simulink model "Simscape_model_Energy"  (R2026a)
settings: Solver=FixedStepAuto  StopTime=8  FixedStep=0.0001
model workspace (MATLAB code in the model file):
  | clear; clc; close all;
values from neighbouring files (symbols this model uses):
  black = partTemplate    [Parameters.m]    (also in Parameters_optimization.m = struct)
  blueBlock = partTemplate    [Parameters.m]    (also in Parameters_optimization.m = struct)
  cyan = partTemplate    [Parameters.m]    (also in Parameters_optimization.m = struct)
  g = 9.81    [Parameters.m]    (also in Parameters_optimization.m)
  greenBeam = partTemplate    [Parameters.m]    (also in Parameters_optimization.m = struct)
  greenBlock = partTemplate    [Parameters.m]    (also in Parameters_optimization.m = struct)
  grey = partTemplate    [Parameters.m]    (also in Parameters_optimization.m = struct)
  IMax = 16    [Parameters.m]    (also in Parameters_optimization.m)
  IMin = -16    [Parameters.m]    (also in Parameters_optimization.m)
  JM = 0.002    [Parameters.m]    (also in Parameters_optimization.m)
  KdA_pos = 1    [Parameters.m]    (also in Parameters_optimization.m = 5066.74)
  KdA_vel = 0    [Parameters.m]    (also in Parameters_optimization.m)
  KdB1_pos = 1    [Parameters.m]    (also in Parameters_optimization.m = 4.04669)
  KdB1_vel = 0    [Parameters.m]    (also in Parameters_optimization.m)
  KdB2_pos = 1    [Parameters.m]    (also in Parameters_optimization.m = 1.06194)
  KdB2_vel = 0    [Parameters.m]    (also in Parameters_optimization.m)
  KdG_pos = 1    [Parameters.m]    (also in Parameters_optimization.m = 1.01282)
  KdG_vel = 0    [Parameters.m]    (also in Parameters_optimization.m)
  KdH_pos = 1    [Parameters.m]    (also in Parameters_optimization.m = 16.6487)
  KdH_vel = 0    [Parameters.m]    (also in Parameters_optimization.m)
  KdI_pos = 1    [Parameters.m]    (also in Parameters_optimization.m = 2.31436)
  KdI_vel = 0    [Parameters.m]    (also in Parameters_optimization.m)
  KiA_pos = 2    [Parameters.m]    (also in Parameters_optimization.m = 1.00755)
  KiA_vel = 5    [Parameters.m]    (also in Parameters_optimization.m)
  KiB1_pos = 30    [Parameters.m]    (also in Parameters_optimization.m = 45.4381)
  KiB1_vel = 10    [Parameters.m]    (also in Parameters_optimization.m)
  KiB2_pos = 20    [Parameters.m]    (also in Parameters_optimization.m = 84.4311)
  KiB2_vel = 5    [Parameters.m]    (also in Parameters_optimization.m)
  KiG_pos = 30    [Parameters.m]    (also in Parameters_optimization.m = 81.5274)
  KiG_vel = 5    [Parameters.m]    (also in Parameters_optimization.m)
  KiH_pos = 10    [Parameters.m]    (also in Parameters_optimization.m = 20739.8)
  KiH_vel = 0    [Parameters.m]    (also in Parameters_optimization.m)
  KiI_pos = 0    [Parameters.m]    (also in Parameters_optimization.m = 1)
  KiI_vel = 0    [Parameters.m]    (also in Parameters_optimization.m)
  KmA = 1.5    [Parameters.m]    (also in Parameters_optimization.m = 1)
  KmB1 = 1.5    [Parameters.m]    (also in Parameters_optimization.m)
  KmB2 = 1.5    [Parameters.m]    (also in Parameters_optimization.m = 1)
  KmG = 0.5    [Parameters.m]    (also in Parameters_optimization.m)
  KmH = 1    [Parameters.m]    (also in Parameters_optimization.m = 0.5)
  KmI = 0.5    [Parameters.m]    (also in Parameters_optimization.m)
  KpA_pos = 150    [Parameters.m]    (also in Parameters_optimization.m = 1588.6)
  KpA_vel = 30    [Parameters.m]    (also in Parameters_optimization.m)
  KpB1_pos = 200    [Parameters.m]    (also in Parameters_optimization.m = 698393)
  KpB1_vel = 30    [Parameters.m]    (also in Parameters_optimization.m)
  KpB2_pos = 150    [Parameters.m]    (also in Parameters_optimization.m = 504375)
  KpB2_vel = 30    [Parameters.m]    (also in Parameters_optimization.m)
  KpG_pos = 100    [Parameters.m]    (also in Parameters_optimization.m = 2817.67)
  KpG_vel = 50    [Parameters.m]    (also in Parameters_optimization.m)
  KpH_pos = 100    [Parameters.m]    (also in Parameters_optimization.m = 12634.3)
  KpH_vel = 20    [Parameters.m]    (also in Parameters_optimization.m)
  KpI_pos = 50    [Parameters.m]    (also in Parameters_optimization.m = 2283.96)
  KpI_vel = 20    [Parameters.m]    (also in Parameters_optimization.m)
  LB1 = 0.8    [Parameters.m]    (also in Parameters_optimization.m)
  LB2 = 0.3    [Parameters.m]    (also in Parameters_optimization.m)
  LB3 = 0.24    [Parameters.m]    (also in Parameters_optimization.m)
  Lblack1 = 0.2    [Parameters.m]    (also in Parameters_optimization.m)
  LC1 = 0.4    [Parameters.m]    (also in Parameters_optimization.m)
  LC2 = 0.225    [Parameters.m]    (also in Parameters_optimization.m)
  LG1 = 0.3    [Parameters.m]    (also in Parameters_optimization.m)
  LG2 = 0.8    [Parameters.m]    (also in Parameters_optimization.m)
  Lgrey1 = 1.175    [Parameters.m]    (also in Parameters_optimization.m)
  lightBlue = partTemplate    [Parameters.m]    (also in Parameters_optimization.m = struct)
  LLB1 = 0.248    [Parameters.m]    (also in Parameters_optimization.m)
  LLB2 = 0.235    [Parameters.m]    (also in Parameters_optimization.m)
  LR1 = 1.05    [Parameters.m]    (also in Parameters_optimization.m)
  LW1 = 1.05    [Parameters.m]    (also in Parameters_optimization.m)
  nA = 200    [Parameters.m]    (also in Parameters_optimization.m = 100)
  nB1 = 200    [Parameters.m]    (also in Parameters_optimization.m = 100)
  nB2 = 200    [Parameters.m]    (also in Parameters_optimization.m)
  nG = 20    [Parameters.m]    (also in Parameters_optimization.m)
  nH = 100    [Parameters.m]    (also in Parameters_optimization.m = 50)
  nI = 20    [Parameters.m]    (also in Parameters_optimization.m)
  omegaFilterA_pos = 60    [Parameters.m]    (also in Parameters_optimization.m)
  omegaFilterA_vel = 60    [Parameters.m]    (also in Parameters_optimization.m)
  omegaFilterB1_pos = 60    [Parameters.m]    (also in Parameters_optimization.m)
  omegaFilterB1_vel = 60    [Parameters.m]    (also in Parameters_optimization.m)
  omegaFilterB2_pos = 60    [Parameters.m]    (also in Parameters_optimization.m)
  omegaFilterB2_vel = 60    [Parameters.m]    (also in Parameters_optimization.m)
  omegaFilterG_pos = 60    [Parameters.m]    (also in Parameters_optimization.m)
  omegaFilterG_vel = 60    [Parameters.m]    (also in Parameters_optimization.m)
  omegaFilterH_pos = 60    [Parameters.m]    (also in Parameters_optimization.m)
  omegaFilterH_vel = 60    [Parameters.m]    (also in Parameters_optimization.m)
  omegaFilterI_pos = 60    [Parameters.m]    (also in Parameters_optimization.m)
  omegaFilterI_vel = 60    [Parameters.m]    (also in Parameters_optimization.m)
  red = partTemplate    [Parameters.m]    (also in Parameters_optimization.m = struct)
  trajCoeff = coeff    [Parameters.m]    (also in Parameters_optimization.m = [2000 500 1600; Path_Planning_Robot.m)
  trajTime = t    [Parameters.m]    (also in Parameters_optimization.m = [0 2 4 6 8]; Path_Planning_Robot.m)
  w = 0.1    [Parameters.m]    (also in Parameters_optimization.m)
  white = partTemplate    [Parameters.m]    (also in Parameters_optimization.m = struct)
undefined symbols (not defined in the file or in its folder): X, Y, Z
libraries: sm_lib x102, nesl_utility x58, simulink x1
(part 4 of 4)

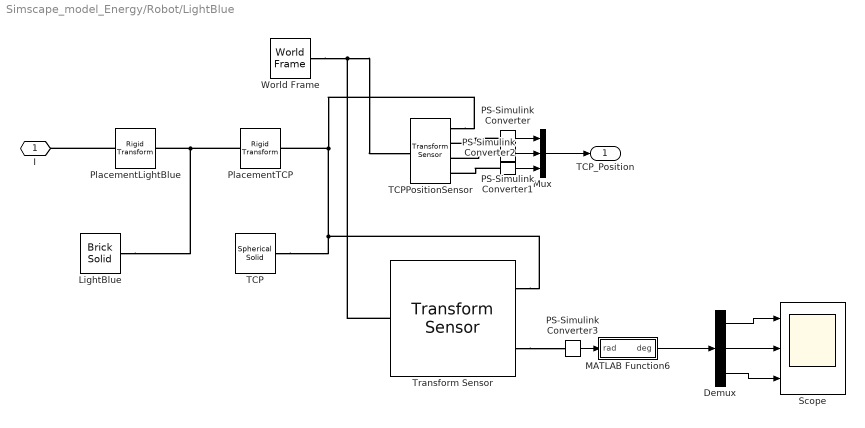
== system Simscape_model_Energy/Robot/LightBlue ==
  Demux : Demux  Outputs=3
  LightBlue : sm_lib/Body Elements/Brick Solid  BrickDimensions=[LLB2 LLB1 LLB1]  BrickDimensionsUnits=m  ExportEntireGeometry=off  InertiaType=Custom  BasedOnType=Density  Density=1000  DensityUnits=kg/m^3  Mass=lightBlue.m  MassUnits=kg  CenterOfMass=[0 0 0]  CenterOfMassUnits=m  MomentsOfInertia=[lightBlue.Ix lightBlue.Iy lightBlue.Iz]  MomentsOfInertiaUnits=kg*m^2  ProductsOfInertia=[0 0 0]  ProductsOfInertiaUnits=kg*m^2  GraphicType=FromGeometry  MarkerShape=Sphere  MarkerSize=10  GraphicVisPropType=SimpleVisualProperties  GraphicDiffuseColor=[0.6667 1 1]  GraphicOpacity=1  GraphicSpecularColor=[0.5 0.5 0.5 1.0]  GraphicAmbientColor=[0.15 0.15 0.15 1.0]  GraphicEmissiveColor=[0.0 0.0 0.0 1.0]  GraphicShininess=75  DoExposeReferenceFrame=on  SerializedFrames=<Frames/>
  MATLAB Function6 : MATLAB Function  TreatAsAtomicUnit=on
  Mux : Mux  Inputs=3
  PS-Simulink Converter{,1..3} (4 alike) : nesl_utility/PS-Simulink Converter  PhysicalDomain=network_engine_domain  SubClassName=ps_output  LeftPortType=input  RightPortType=output  PseudoPeriodic=off  Frequencies=[]  VectorFormat=inherit  Unit=inherit  AffineConversion=off
  PlacementLightBlue : sm_lib/Frames and Transforms/Rigid Transform  RotationMethod=RotationSequence  FollAlignAxisA=+X  BaseAlignAxisA=+Y  FollAlignAxisB=+Y  BaseAlignAxisB=+Z  RotationStandardAxis=+Z  RotationAngle=0  RotationAngleUnits=deg  RotationArbitraryAxis=[0 0 1]  RotationSequenceAxes=FollowerAxes  RotationSequence=XYZ  RotationSequenceAngles=[90 0 90]  RotationSequenceAnglesUnits=deg  RotationMatrix=[1 0 0;0 1 0;0 0 1]  Quaternion=[1 0 0 0]  TranslationMethod=Cartesian  TranslationCartesianOffset=[0 LLB1/2 LLB2/2]  TranslationCartesianOffsetUnits=m  TranslationStandardAxis=+Z  TranslationStandardOffset=0  TranslationStandardOffsetUnits=m  TranslationROffset=0  TranslationROffsetUnits=m  TranslationThetaOffset=0  TranslationThetaOffsetUnits=deg  TranslationZOffset=0  TranslationZOffsetUnits=m
  PlacementTCP : sm_lib/Frames and Transforms/Rigid Transform  RotationMethod=None  FollAlignAxisA=+X  BaseAlignAxisA=+Y  FollAlignAxisB=+Y  BaseAlignAxisB=+Z  RotationStandardAxis=+Z  RotationAngle=0  RotationAngleUnits=deg  RotationArbitraryAxis=[0 0 1]  RotationSequenceAxes=FollowerAxes  RotationSequence=XYZ  RotationSequenceAngles=[0 0 0]  RotationSequenceAnglesUnits=deg  RotationMatrix=[1 0 0;0 1 0;0 0 1]  Quaternion=[1 0 0 0]  TranslationMethod=Cartesian  TranslationCartesianOffset=[LLB1/2 0 -LLB2/2]  TranslationCartesianOffsetUnits=m  TranslationStandardAxis=+Z  TranslationStandardOffset=0  TranslationStandardOffsetUnits=m  TranslationROffset=0  TranslationROffsetUnits=m  TranslationThetaOffset=0  TranslationThetaOffsetUnits=deg  TranslationZOffset=0  TranslationZOffsetUnits=m
  Scope : Scope  NumInputPorts=3
      settings: ActiveDisplayYMinimum=-0.24123535125414011  ActiveDisplayYMaximum=0.21681941956598327  DataLoggingVariableName=ScopeData9
  TCP : sm_lib/Body Elements/Spherical Solid  SphereRadius=w  SphereRadiusUnits=m  ExportEntireGeometry=off  InertiaType=CalculateFromGeometry  BasedOnType=Mass  Density=0  DensityUnits=kg/m^3  Mass=0  MassUnits=kg  CenterOfMass=[0 0 0]  CenterOfMassUnits=m  MomentsOfInertia=[1 1 1]  MomentsOfInertiaUnits=kg*m^2  ProductsOfInertia=[0 0 0]  ProductsOfInertiaUnits=kg*m^2  GraphicType=FromGeometry  MarkerShape=Sphere  MarkerSize=10  GraphicVisPropType=SimpleVisualProperties  GraphicDiffuseColor=[1 0 1]  GraphicOpacity=1  GraphicSpecularColor=[0.5 0.5 0.5 1.0]  GraphicAmbientColor=[0.15 0.15 0.15 1.0]  GraphicEmissiveColor=[0.0 0.0 0.0 1.0]  GraphicShininess=75  DoExposeReferenceFrame=on  SerializedFrames=<Frames/>
  TCPPositionSensor : sm_lib/Frames and Transforms/Transform Sensor  MeasurementFrame=World  RotationSequence=XYX  SenseAngle=off  SenseAxis=off  SenseQ=off  SenseR=off  SenseRotationSequence=off  SenseOmegaX=off  SenseOmegaY=off  SenseOmegaZ=off  SenseOmega=off  SenseQDot=off  SenseRDot=off  SenseRotationSequenceDot=off  SenseAlphaX=off  SenseAlphaY=off  SenseAlphaZ=off  SenseAlpha=off  SenseQDDot=off  SenseRDDot=off  SenseX=on  SenseY=on  SenseZ=on  SenseXYZ=off  SenseRad=off  SenseAzim=off  SenseDist=off  SenseInc=off  SenseXDot=off  SenseYDot=off  SenseZDot=off  SenseXYZDot=off  SenseRadDot=off  SenseAzimDot=off  SenseDistDot=off  SenseIncDot=off  SenseXDDot=off  SenseYDDot=off  SenseZDDot=off  SenseXYZDDot=off  SenseRadDDot=off  SenseAzimDDot=off  SenseDistDDot=off  SenseIncDDot=off
  Transform Sensor : sm_lib/Frames and Transforms/Transform Sensor  MeasurementFrame=World  RotationSequence=XYZ  SenseAngle=off  SenseAxis=off  SenseQ=off  SenseR=off  SenseRotationSequence=on  SenseOmegaX=off  SenseOmegaY=off  SenseOmegaZ=off  SenseOmega=off  SenseQDot=off  SenseRDot=off  SenseRotationSequenceDot=off  SenseAlphaX=off  SenseAlphaY=off  SenseAlphaZ=off  SenseAlpha=off  SenseQDDot=off  SenseRDDot=off  SenseX=off  SenseY=off  SenseZ=off  SenseXYZ=off  SenseRad=off  SenseAzim=off  SenseDist=off  SenseInc=off  SenseXDot=off  SenseYDot=off  SenseZDot=off  SenseXYZDot=off  SenseRadDot=off  SenseAzimDot=off  SenseDistDot=off  SenseIncDot=off  SenseXDDot=off  SenseYDDot=off  SenseZDDot=off  SenseXYZDDot=off  SenseRadDDot=off  SenseAzimDDot=off  SenseDistDDot=off  SenseIncDDot=off
  World Frame : sm_lib/Frames and Transforms/World Frame
  I : PMIOPort  Side=Left
  TCP_Position : Outport
  wires:
  PS-Simulink Converter2/1 -> Mux/3
  PS-Simulink Converter1/1 -> Mux/2
  PS-Simulink Converter/1 -> Mux/1
  Mux/1 -> TCP_Position/1
  PS-Simulink Converter3/1 -> MATLAB Function6/1(rad)
  Demux/1 -> Scope/1
  Demux/2 -> Scope/2
  Demux/3 -> Scope/3
  MATLAB Function6/1(deg) -> Demux/1
  connections:
  TCP/RConn1 -- TCPPositionSensor/RConn1 -- PlacementTCP/RConn1 -- Transform Sensor/RConn1
  LightBlue/RConn1 -- PlacementTCP/LConn1 -- PlacementLightBlue/RConn1
  PlacementLightBlue/LConn1 -- I/RConn1
  PS-Simulink Converter/LConn1 -- TCPPositionSensor/RConn2
  PS-Simulink Converter1/LConn1 -- TCPPositionSensor/RConn3
  PS-Simulink Converter2/LConn1 -- TCPPositionSensor/RConn4
  World Frame/RConn1 -- Transform Sensor/LConn1 -- TCPPositionSensor/LConn1
  Transform Sensor/RConn2 -- PS-Simulink Converter3/LConn1

== system Simscape_model_Energy/Robot/Red ==
  PlacementJ3 : sm_lib/Frames and Transforms/Rigid Transform  RotationMethod=None  FollAlignAxisA=+X  BaseAlignAxisA=+Y  FollAlignAxisB=+Y  BaseAlignAxisB=+Z  RotationStandardAxis=+Z  RotationAngle=0  RotationAngleUnits=deg  RotationArbitraryAxis=[0 0 1]  RotationSequenceAxes=FollowerAxes  RotationSequence=XYX  RotationSequenceAngles=[0 0 0]  RotationSequenceAnglesUnits=deg  RotationMatrix=[1 0 0;0 1 0;0 0 1]  Quaternion=[1 0 0 0]  TranslationMethod=Cartesian  TranslationCartesianOffset=[-LR1/2 0 0]  TranslationCartesianOffsetUnits=m  TranslationStandardAxis=+Z  TranslationStandardOffset=0  TranslationStandardOffsetUnits=m  TranslationROffset=0  TranslationROffsetUnits=m  TranslationThetaOffset=0  TranslationThetaOffsetUnits=deg  TranslationZOffset=0  TranslationZOffsetUnits=m
  PlacementRed : sm_lib/Frames and Transforms/Rigid Transform  RotationMethod=RotationSequence  FollAlignAxisA=+X  BaseAlignAxisA=+Y  FollAlignAxisB=+Y  BaseAlignAxisB=+Z  RotationStandardAxis=+Z  RotationAngle=0  RotationAngleUnits=deg  RotationArbitraryAxis=[0 0 1]  RotationSequenceAxes=FollowerAxes  RotationSequence=XYZ  RotationSequenceAngles=[0 0 -90]  RotationSequenceAnglesUnits=deg  RotationMatrix=[1 0 0;0 1 0;0 0 1]  Quaternion=[1 0 0 0]  TranslationMethod=Cartesian  TranslationCartesianOffset=[-LR1/2 0 0]  TranslationCartesianOffsetUnits=m  TranslationStandardAxis=+Z  TranslationStandardOffset=0  TranslationStandardOffsetUnits=m  TranslationROffset=0  TranslationROffsetUnits=m  TranslationThetaOffset=0  TranslationThetaOffsetUnits=deg  TranslationZOffset=0  TranslationZOffsetUnits=m
  Red : sm_lib/Body Elements/Brick Solid  BrickDimensions=[LR1 w w]  BrickDimensionsUnits=m  ExportEntireGeometry=off  InertiaType=Custom  BasedOnType=Density  Density=1000  DensityUnits=kg/m^3  Mass=red.m  MassUnits=kg  CenterOfMass=[0 0 0]  CenterOfMassUnits=m  MomentsOfInertia=[red.Ix red.Iy red.Iz]  MomentsOfInertiaUnits=kg*m^2  ProductsOfInertia=[0 0 0]  ProductsOfInertiaUnits=kg*m^2  GraphicType=FromGeometry  MarkerShape=Sphere  MarkerSize=10  GraphicVisPropType=SimpleVisualProperties  GraphicDiffuseColor=[1 0 0]  GraphicOpacity=1  GraphicSpecularColor=[0.5 0.5 0.5 1.0]  GraphicAmbientColor=[0.15 0.15 0.15 1.0]  GraphicEmissiveColor=[0.0 0.0 0.0 1.0]  GraphicShininess=75  DoExposeReferenceFrame=on  SerializedFrames=<Frames/>
  E : PMIOPort  Side=Left
  B : PMIOPort  Port=2  Side=Right
  connections:
  B/RConn1 -- PlacementRed/RConn1
  PlacementRed/LConn1 -- PlacementJ3/RConn1 -- Red/RConn1
  E/RConn1 -- PlacementJ3/LConn1

== system Simscape_model_Energy/Robot/Subsystem ==
  PlacementF : sm_lib/Frames and Transforms/Rigid Transform  RotationMethod=None  FollAlignAxisA=+X  BaseAlignAxisA=+Y  FollAlignAxisB=+Y  BaseAlignAxisB=+Z  RotationStandardAxis=+Z  RotationAngle=0  RotationAngleUnits=deg  RotationArbitraryAxis=[0 0 1]  RotationSequenceAxes=FollowerAxes  RotationSequence=XYX  RotationSequenceAngles=[0 0 0]  RotationSequenceAnglesUnits=deg  RotationMatrix=[1 0 0;0 1 0;0 0 1]  Quaternion=[1 0 0 0]  TranslationMethod=Cartesian  TranslationCartesianOffset=[LW1/2 0 0]  TranslationCartesianOffsetUnits=m  TranslationStandardAxis=+Z  TranslationStandardOffset=0  TranslationStandardOffsetUnits=m  TranslationROffset=0  TranslationROffsetUnits=m  TranslationThetaOffset=0  TranslationThetaOffsetUnits=deg  TranslationZOffset=0  TranslationZOffsetUnits=m
  PlacementWhite : sm_lib/Frames and Transforms/Rigid Transform  RotationMethod=RotationSequence  FollAlignAxisA=+X  BaseAlignAxisA=+Y  FollAlignAxisB=+Y  BaseAlignAxisB=+Z  RotationStandardAxis=+Z  RotationAngle=0  RotationAngleUnits=deg  RotationArbitraryAxis=[0 0 1]  RotationSequenceAxes=FollowerAxes  RotationSequence=XYZ  RotationSequenceAngles=[0 0 90]  RotationSequenceAnglesUnits=deg  RotationMatrix=[1 0 0;0 1 0;0 0 1]  Quaternion=[1 0 0 0]  TranslationMethod=Cartesian  TranslationCartesianOffset=[LW1/2 0 0]  TranslationCartesianOffsetUnits=m  TranslationStandardAxis=+Z  TranslationStandardOffset=0  TranslationStandardOffsetUnits=m  TranslationROffset=0  TranslationROffsetUnits=m  TranslationThetaOffset=0  TranslationThetaOffsetUnits=deg  TranslationZOffset=0  TranslationZOffsetUnits=m
  White : sm_lib/Body Elements/Brick Solid  BrickDimensions=[LW1 w w]  BrickDimensionsUnits=m  ExportEntireGeometry=off  InertiaType=Custom  BasedOnType=Density  Density=1000  DensityUnits=kg/m^3  Mass=white.m  MassUnits=kg  CenterOfMass=[0 0 0]  CenterOfMassUnits=m  MomentsOfInertia=[white.Ix white.Iy white.Iz]  MomentsOfInertiaUnits=kg*m^2  ProductsOfInertia=[0 0 0]  ProductsOfInertiaUnits=kg*m^2  GraphicType=FromGeometry  MarkerShape=Sphere  MarkerSize=10  GraphicVisPropType=SimpleVisualProperties  GraphicDiffuseColor=[1 1 1]  GraphicOpacity=1  GraphicSpecularColor=[0.5 0.5 0.5 1.0]  GraphicAmbientColor=[0.15 0.15 0.15 1.0]  GraphicEmissiveColor=[0.0 0.0 0.0 1.0]  GraphicShininess=75  DoExposeReferenceFrame=on  SerializedFrames=<Frames/>
  F : PMIOPort  Side=Left
  D : PMIOPort  Port=2  Side=Right
  connections:
  White/RConn1 -- PlacementF/RConn1 -- PlacementWhite/LConn1
  F/RConn1 -- PlacementF/LConn1
  PlacementWhite/RConn1 -- D/RConn1

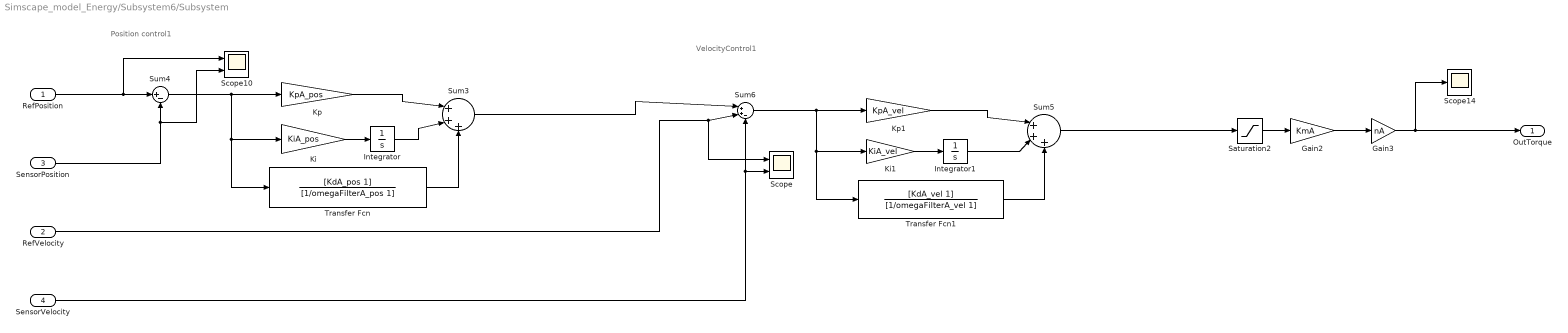
== system Simscape_model_Energy/Subsystem6/Subsystem ==
  note: VelocityControl1
  note: Position control1
  RefPosition : Inport
  RefVelocity : Inport  Port=2
  SensorPosition : Inport  Port=3
  SensorVelocity : Inport  Port=4
  Gain2 : Gain  Gain=KmA
  Gain3 : Gain  Gain=nA
  Integrator : Integrator
  Integrator1 : Integrator
  Ki : Gain  Gain=KiA_pos
  Ki1 : Gain  Gain=KiA_vel
  Kp : Gain  Gain=KpA_pos
  Kp1 : Gain  Gain=KpA_vel
  Saturation2 : Saturate  UpperLimit=IMax  LowerLimit=IMin
  Scope : Scope  NumInputPorts=2
      settings: ActiveDisplayYMinimum=-0.68131991741481623  ActiveDisplayYMaximum=0.75407267778393594  DataLoggingVariableName=ScopeData11
  Scope10 : Scope  NumInputPorts=2
      settings: ActiveDisplayYMinimum=-0.35494111155863695  ActiveDisplayYMaximum=-0.26838705536276919  DataLoggingVariableName=ScopeData6
  Scope14 : Scope
      settings: ActiveDisplayYMinimum=-1  ActiveDisplayYMaximum=1  DataLoggingVariableName=ScopeData12
  Sum3 : Sum  Inputs=|+++
  Sum4 : Sum  Inputs=|+-
  Sum5 : Sum  Inputs=|+++
  Sum6 : Sum  Inputs=|++-
  Transfer Fcn : TransferFcn  Numerator=[KdA_pos 1]  Denominator=[1/omegaFilterA_pos 1]
  Transfer Fcn1 : TransferFcn  Numerator=[KdA_vel 1]  Denominator=[1/omegaFilterA_vel 1]
  OutTorque : Outport
  wires:
  Gain2/1 -> Gain3/1
  Sum6/1 -> Kp1/1, Transfer Fcn1/1, Ki1/1
  Gain3/1 -> OutTorque/1, Scope14/1
  RefPosition/1 -> Scope10/1, Sum4/1
  Transfer Fcn/1 -> Sum3/3
  RefVelocity/1 -> Scope/1, Sum6/2
  SensorVelocity/1 -> Sum6/3, Scope/2
  Ki1/1 -> Integrator1/1
  Saturation2/1 -> Gain2/1
  SensorPosition/1 -> Scope10/2, Sum4/2
  Kp1/1 -> Sum5/1
  Sum3/1 -> Sum6/1
  Ki/1 -> Integrator/1
  Sum4/1 -> Kp/1, Transfer Fcn/1, Ki/1
  Integrator/1 -> Sum3/2
  Kp/1 -> Sum3/1
  Sum5/1 -> Saturation2/1
  Transfer Fcn1/1 -> Sum5/3
  Integrator1/1 -> Sum5/2

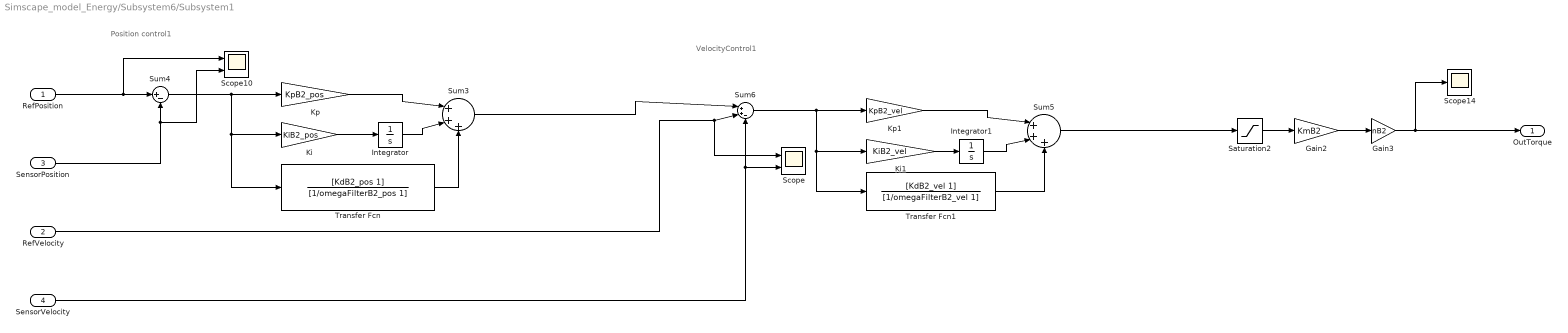
== system Simscape_model_Energy/Subsystem6/Subsystem1 ==
  note: VelocityControl1
  note: Position control1
  RefPosition : Inport
  RefVelocity : Inport  Port=2
  SensorPosition : Inport  Port=3
  SensorVelocity : Inport  Port=4
  Gain2 : Gain  Gain=KmB2
  Gain3 : Gain  Gain=nB2
  Integrator : Integrator
  Integrator1 : Integrator
  Ki : Gain  Gain=KiB2_pos
  Ki1 : Gain  Gain=KiB2_vel
  Kp : Gain  Gain=KpB2_pos
  Kp1 : Gain  Gain=KpB2_vel
  Saturation2 : Saturate  UpperLimit=IMax  LowerLimit=IMin
  Scope : Scope  NumInputPorts=2
      settings: ActiveDisplayYMinimum=-0.67693096974028455  ActiveDisplayYMaximum=0.584259870877825  DataLoggingVariableName=ScopeData13
  Scope10 : Scope  NumInputPorts=2
      settings: ActiveDisplayYMinimum=-0.094492964646165772  ActiveDisplayYMaximum=0.8532084350466248  DataLoggingVariableName=ScopeData6
  Scope14 : Scope
      settings: ActiveDisplayYMinimum=-591.57740919857179  ActiveDisplayYMaximum=3621.2863787998413  DataLoggingVariableName=ScopeData12
  Sum3 : Sum  Inputs=|+++
  Sum4 : Sum  Inputs=|+-
  Sum5 : Sum  Inputs=|+++
  Sum6 : Sum  Inputs=|++-
  Transfer Fcn : TransferFcn  Numerator=[KdB2_pos 1]  Denominator=[1/omegaFilterB2_pos 1]
  Transfer Fcn1 : TransferFcn  Numerator=[KdB2_vel 1]  Denominator=[1/omegaFilterB2_vel 1]
  OutTorque : Outport
  wires:
  Gain2/1 -> Gain3/1
  Sum6/1 -> Kp1/1, Transfer Fcn1/1, Ki1/1
  Gain3/1 -> OutTorque/1, Scope14/1
  RefPosition/1 -> Scope10/1, Sum4/1
  Transfer Fcn/1 -> Sum3/3
  RefVelocity/1 -> Scope/1, Sum6/2
  SensorVelocity/1 -> Sum6/3, Scope/2
  Ki1/1 -> Integrator1/1
  Saturation2/1 -> Gain2/1
  SensorPosition/1 -> Scope10/2, Sum4/2
  Kp1/1 -> Sum5/1
  Sum3/1 -> Sum6/1
  Ki/1 -> Integrator/1
  Sum4/1 -> Kp/1, Transfer Fcn/1, Ki/1
  Integrator/1 -> Sum3/2
  Kp/1 -> Sum3/1
  Sum5/1 -> Saturation2/1
  Transfer Fcn1/1 -> Sum5/3
  Integrator1/1 -> Sum5/2

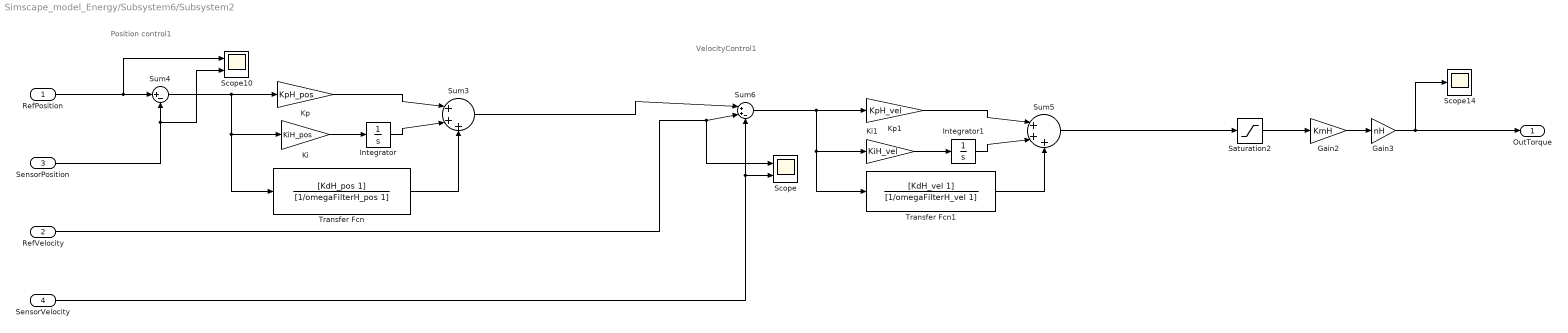
== system Simscape_model_Energy/Subsystem6/Subsystem2 ==
  note: VelocityControl1
  note: Position control1
  RefPosition : Inport
  RefVelocity : Inport  Port=2
  SensorPosition : Inport  Port=3
  SensorVelocity : Inport  Port=4
  Gain2 : Gain  Gain=KmH
  Gain3 : Gain  Gain=nH
  Integrator : Integrator
  Integrator1 : Integrator
  Ki : Gain  Gain=KiH_pos
  Ki1 : Gain  Gain=KiH_vel
  Kp : Gain  Gain=KpH_pos
  Kp1 : Gain  Gain=KpH_vel
  Saturation2 : Saturate  UpperLimit=IMax  LowerLimit=IMin
  Scope : Scope  NumInputPorts=2
      settings: ActiveDisplayYMinimum=-0.25589923136738535  ActiveDisplayYMaximum=0.25103879002205542  DataLoggingVariableName=ScopeData15
  Scope10 : Scope  NumInputPorts=2
      settings: ActiveDisplayYMinimum=-0.5862610022981225  ActiveDisplayYMaximum=-0.12292535976810215  DataLoggingVariableName=ScopeData6
  Scope14 : Scope
      settings: ActiveDisplayYMinimum=-1  ActiveDisplayYMaximum=1  DataLoggingVariableName=ScopeData12
  Sum3 : Sum  Inputs=|+++
  Sum4 : Sum  Inputs=|+-
  Sum5 : Sum  Inputs=|+++
  Sum6 : Sum  Inputs=|++-
  Transfer Fcn : TransferFcn  Numerator=[KdH_pos 1]  Denominator=[1/omegaFilterH_pos 1]
  Transfer Fcn1 : TransferFcn  Numerator=[KdH_vel 1]  Denominator=[1/omegaFilterH_vel 1]
  OutTorque : Outport
  wires:
  Gain2/1 -> Gain3/1
  Sum6/1 -> Kp1/1, Transfer Fcn1/1, Ki1/1
  Gain3/1 -> OutTorque/1, Scope14/1
  RefPosition/1 -> Scope10/1, Sum4/1
  Transfer Fcn/1 -> Sum3/3
  RefVelocity/1 -> Scope/1, Sum6/2
  SensorVelocity/1 -> Scope/2, Sum6/3
  Ki1/1 -> Integrator1/1
  Saturation2/1 -> Gain2/1
  SensorPosition/1 -> Scope10/2, Sum4/2
  Kp1/1 -> Sum5/1
  Sum3/1 -> Sum6/1
  Ki/1 -> Integrator/1
  Sum4/1 -> Kp/1, Transfer Fcn/1, Ki/1
  Integrator/1 -> Sum3/2
  Kp/1 -> Sum3/1
  Sum5/1 -> Saturation2/1
  Transfer Fcn1/1 -> Sum5/3
  Integrator1/1 -> Sum5/2

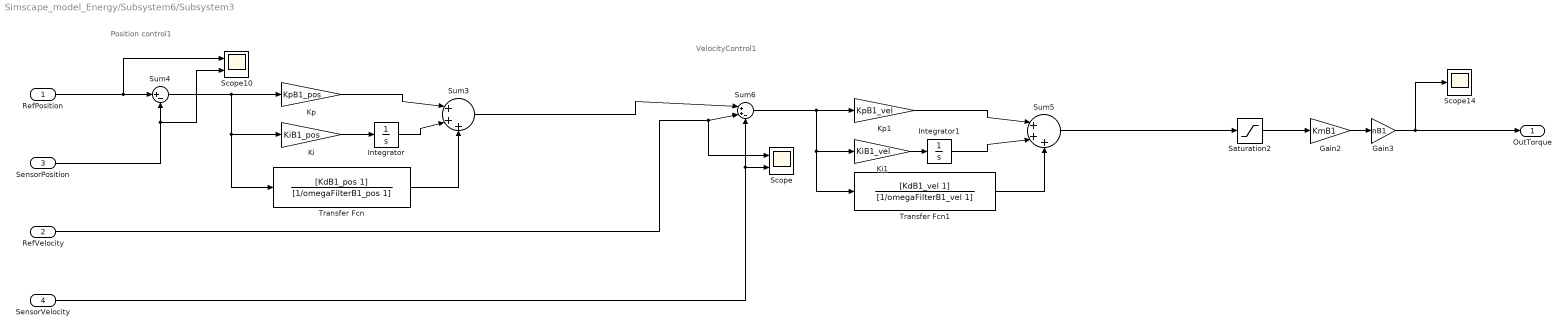
== system Simscape_model_Energy/Subsystem6/Subsystem3 ==
  note: VelocityControl1
  note: Position control1
  RefPosition : Inport
  RefVelocity : Inport  Port=2
  SensorPosition : Inport  Port=3
  SensorVelocity : Inport  Port=4
  Gain2 : Gain  Gain=KmB1
  Gain3 : Gain  Gain=nB1
  Integrator : Integrator
  Integrator1 : Integrator
  Ki : Gain  Gain=KiB1_pos
  Ki1 : Gain  Gain=KiB1_vel
  Kp : Gain  Gain=KpB1_pos
  Kp1 : Gain  Gain=KpB1_vel
  Saturation2 : Saturate  UpperLimit=IMax  LowerLimit=IMin
  Scope : Scope  NumInputPorts=2
      settings: ActiveDisplayYMinimum=-1  ActiveDisplayYMaximum=1  DataLoggingVariableName=ScopeData10
  Scope10 : Scope  NumInputPorts=2
      settings: ActiveDisplayYMinimum=-0.22429334288555461  ActiveDisplayYMaximum=0.086095716929386459  DataLoggingVariableName=ScopeData6
  Scope14 : Scope
      settings: ActiveDisplayYMinimum=-1  ActiveDisplayYMaximum=1  DataLoggingVariableName=ScopeData12
  Sum3 : Sum  Inputs=|+++
  Sum4 : Sum  Inputs=|+-
  Sum5 : Sum  Inputs=|+++
  Sum6 : Sum  Inputs=|++-
  Transfer Fcn : TransferFcn  Numerator=[KdB1_pos 1]  Denominator=[1/omegaFilterB1_pos 1]
  Transfer Fcn1 : TransferFcn  Numerator=[KdB1_vel 1]  Denominator=[1/omegaFilterB1_vel 1]
  OutTorque : Outport
  wires:
  Gain2/1 -> Gain3/1
  Sum6/1 -> Kp1/1, Transfer Fcn1/1, Ki1/1
  Gain3/1 -> OutTorque/1, Scope14/1
  RefPosition/1 -> Scope10/1, Sum4/1
  Transfer Fcn/1 -> Sum3/3
  RefVelocity/1 -> Scope/1, Sum6/2
  SensorVelocity/1 -> Scope/2, Sum6/3
  Ki1/1 -> Integrator1/1
  Saturation2/1 -> Gain2/1
  SensorPosition/1 -> Scope10/2, Sum4/2
  Kp1/1 -> Sum5/1
  Sum3/1 -> Sum6/1
  Ki/1 -> Integrator/1
  Sum4/1 -> Kp/1, Transfer Fcn/1, Ki/1
  Integrator/1 -> Sum3/2
  Kp/1 -> Sum3/1
  Sum5/1 -> Saturation2/1
  Transfer Fcn1/1 -> Sum5/3
  Integrator1/1 -> Sum5/2

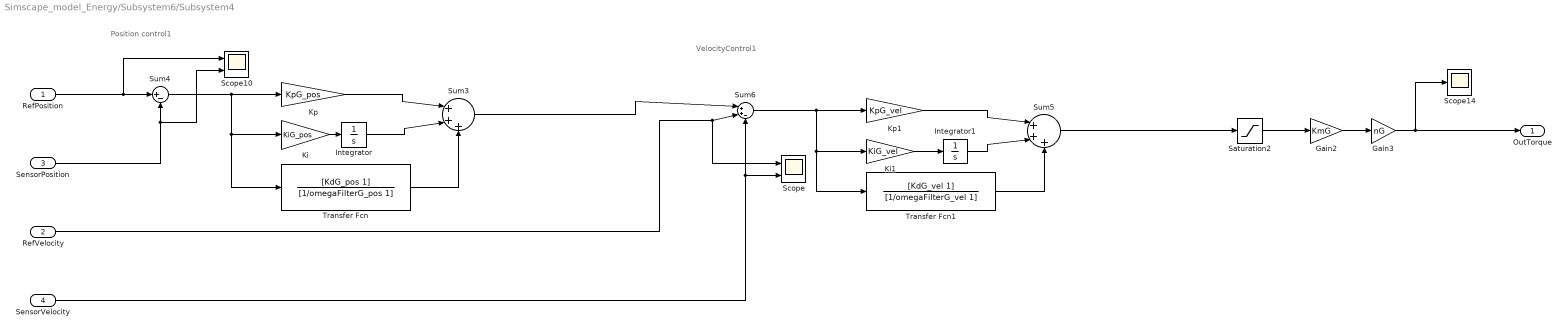
== system Simscape_model_Energy/Subsystem6/Subsystem4 ==
  note: VelocityControl1
  note: Position control1
  RefPosition : Inport
  RefVelocity : Inport  Port=2
  SensorPosition : Inport  Port=3
  SensorVelocity : Inport  Port=4
  Gain2 : Gain  Gain=KmG
  Gain3 : Gain  Gain=nG
  Integrator : Integrator
  Integrator1 : Integrator
  Ki : Gain  Gain=KiG_pos
  Ki1 : Gain  Gain=KiG_vel
  Kp : Gain  Gain=KpG_pos
  Kp1 : Gain  Gain=KpG_vel
  Saturation2 : Saturate  UpperLimit=IMax  LowerLimit=IMin
  Scope : Scope  NumInputPorts=2
      settings: ActiveDisplayYMinimum=-1.9347621453136528  ActiveDisplayYMaximum=3.815265459937685  DataLoggingVariableName=ScopeData14
  Scope10 : Scope  NumInputPorts=2
      settings: ActiveDisplayYMinimum=-0.78991792288648721  ActiveDisplayYMaximum=1.2637375123361299  DataLoggingVariableName=ScopeData6
  Scope14 : Scope
      settings: ActiveDisplayYMinimum=-1  ActiveDisplayYMaximum=1  DataLoggingVariableName=ScopeData12
  Sum3 : Sum  Inputs=|+++
  Sum4 : Sum  Inputs=|+-
  Sum5 : Sum  Inputs=|+++
  Sum6 : Sum  Inputs=|++-
  Transfer Fcn : TransferFcn  Numerator=[KdG_pos 1]  Denominator=[1/omegaFilterG_pos 1]
  Transfer Fcn1 : TransferFcn  Numerator=[KdG_vel 1]  Denominator=[1/omegaFilterG_vel 1]
  OutTorque : Outport
  wires:
  Gain2/1 -> Gain3/1
  Sum6/1 -> Kp1/1, Transfer Fcn1/1, Ki1/1
  Gain3/1 -> OutTorque/1, Scope14/1
  RefPosition/1 -> Scope10/1, Sum4/1
  Transfer Fcn/1 -> Sum3/3
  RefVelocity/1 -> Scope/1, Sum6/2
  SensorVelocity/1 -> Scope/2, Sum6/3
  Ki1/1 -> Integrator1/1
  Saturation2/1 -> Gain2/1
  SensorPosition/1 -> Scope10/2, Sum4/2
  Kp1/1 -> Sum5/1
  Sum3/1 -> Sum6/1
  Ki/1 -> Integrator/1
  Sum4/1 -> Kp/1, Transfer Fcn/1, Ki/1
  Integrator/1 -> Sum3/2
  Kp/1 -> Sum3/1
  Sum5/1 -> Saturation2/1
  Transfer Fcn1/1 -> Sum5/3
  Integrator1/1 -> Sum5/2

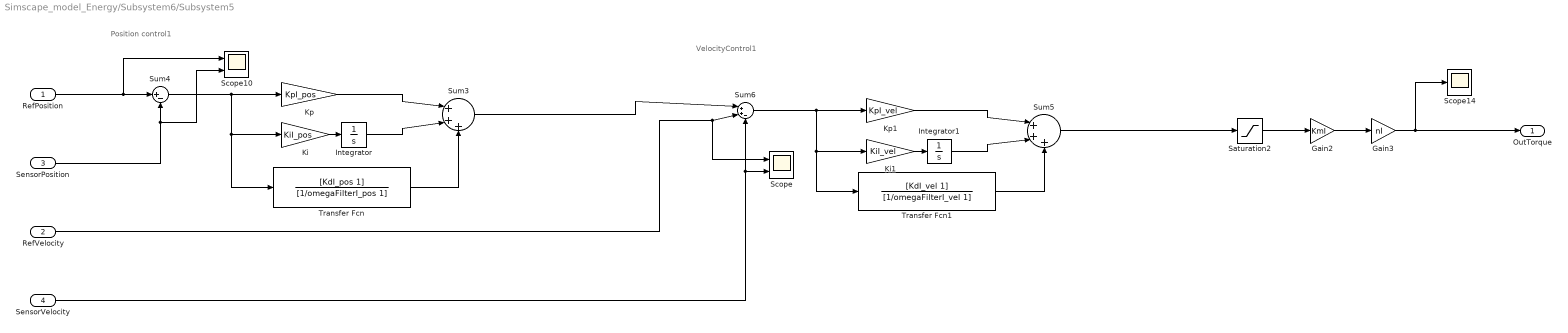
== system Simscape_model_Energy/Subsystem6/Subsystem5 ==
  note: VelocityControl1
  note: Position control1
  RefPosition : Inport
  RefVelocity : Inport  Port=2
  SensorPosition : Inport  Port=3
  SensorVelocity : Inport  Port=4
  Gain2 : Gain  Gain=KmI
  Gain3 : Gain  Gain=nI
  Integrator : Integrator
  Integrator1 : Integrator
  Ki : Gain  Gain=KiI_pos
  Ki1 : Gain  Gain=KiI_vel
  Kp : Gain  Gain=KpI_pos
  Kp1 : Gain  Gain=KpI_vel
  Saturation2 : Saturate  UpperLimit=IMax  LowerLimit=IMin
  Scope : Scope  NumInputPorts=2
      settings: ActiveDisplayYMinimum=-1.3827903663457835  ActiveDisplayYMaximum=2.8017226230223664  DataLoggingVariableName=ScopeData16
  Scope10 : Scope  NumInputPorts=2
      settings: ActiveDisplayYMinimum=-0.72126082385284929  ActiveDisplayYMaximum=1.222924885831816  DataLoggingVariableName=ScopeData6
  Scope14 : Scope
      settings: ActiveDisplayYMinimum=-1  ActiveDisplayYMaximum=1  DataLoggingVariableName=ScopeData12
  Sum3 : Sum  Inputs=|+++
  Sum4 : Sum  Inputs=|+-
  Sum5 : Sum  Inputs=|+++
  Sum6 : Sum  Inputs=|++-
  Transfer Fcn : TransferFcn  Numerator=[KdI_pos 1]  Denominator=[1/omegaFilterI_pos 1]
  Transfer Fcn1 : TransferFcn  Numerator=[KdI_vel 1]  Denominator=[1/omegaFilterI_vel 1]
  OutTorque : Outport
  wires:
  Gain2/1 -> Gain3/1
  Sum6/1 -> Kp1/1, Transfer Fcn1/1, Ki1/1
  Gain3/1 -> OutTorque/1, Scope14/1
  RefPosition/1 -> Scope10/1, Sum4/1
  Transfer Fcn/1 -> Sum3/3
  RefVelocity/1 -> Scope/1, Sum6/2
  SensorVelocity/1 -> Scope/2, Sum6/3
  Ki1/1 -> Integrator1/1
  Saturation2/1 -> Gain2/1
  SensorPosition/1 -> Scope10/2, Sum4/2
  Kp1/1 -> Sum5/1
  Sum3/1 -> Sum6/1
  Ki/1 -> Integrator/1
  Sum4/1 -> Kp/1, Transfer Fcn/1, Ki/1
  Integrator/1 -> Sum3/2
  Kp/1 -> Sum3/1
  Sum5/1 -> Saturation2/1
  Transfer Fcn1/1 -> Sum5/3
  Integrator1/1 -> Sum5/2

== matlab function Simscape_model_Energy/Subsystem1/MATLAB Function7 ==
  data: torque input; P_motoring output; angularVelocity input; P_generating output
function [P_motoring, P_generating] = fcn(torque, angularVelocity)

if (torque <= 0 && angularVelocity < 0) || (torque >= 0 && angularVelocity > 0)
    P_motoring = torque * angularVelocity;
    P_generating = 0;
else
    P_generating = abs(torque * angularVelocity);
    P_motoring = 0;
end

== matlab function Simscape_model_Energy/Subsystem2/MATLAB Function7 ==
  data: torque input; P_motoring output; angularVelocity input; P_generating output
function [P_motoring, P_generating] = fcn(torque, angularVelocity)

if (torque <= 0 && angularVelocity < 0) || (torque >= 0 && angularVelocity > 0)
    P_motoring = torque * angularVelocity;
    P_generating = 0;
else
    P_generating = abs(torque * angularVelocity);
    P_motoring = 0;
end

== matlab function Simscape_model_Energy/Subsystem3/MATLAB Function7 ==
  data: torque input; P_motoring output; angularVelocity input; P_generating output
function [P_motoring, P_generating] = fcn(torque, angularVelocity)

if (torque <= 0 && angularVelocity < 0) || (torque >= 0 && angularVelocity > 0)
    P_motoring = torque * angularVelocity;
    P_generating = 0;
else
    P_generating = abs(torque * angularVelocity);
    P_motoring = 0;
end

== matlab function Simscape_model_Energy/Subsystem4/MATLAB Function7 ==
  data: torque input; P_motoring output; angularVelocity input; P_generating output
function [P_motoring, P_generating] = fcn(torque, angularVelocity)

if (torque <= 0 && angularVelocity < 0) || (torque >= 0 && angularVelocity > 0)
    P_motoring = torque * angularVelocity;
    P_generating = 0;
else
    P_generating = abs(torque * angularVelocity);
    P_motoring = 0;
end

== matlab function Simscape_model_Energy/Subsystem5/MATLAB Function7 ==
  data: torque input; P_motoring output; angularVelocity input; P_generating output
function [P_motoring, P_generating] = fcn(torque, angularVelocity)

if (torque <= 0 && angularVelocity < 0) || (torque >= 0 && angularVelocity > 0)
    P_motoring = torque * angularVelocity;
    P_generating = 0;
else
    P_generating = abs(torque * angularVelocity);
    P_motoring = 0;
end

== matlab function Simscape_model_Energy/MATLAB Function1 ==
  data: u input; y output
function y = fcn(u)

y = u;

== matlab function Simscape_model_Energy/Trajectory/MATLAB Function ==
  data: x output; t input; y output; z output; trajCoeff input; trajTime input
function [x, y, z] = trajectory(t, trajCoeff, trajTime)
 
% Definer utganger
x = 0.0;
y = 0.0;
z = 0.0;
 
% Begrens tiden
t = max(trajTime(1), min(t, trajTime(5)));
 
% Beregn posisjon for riktig tidsintervall
if t <= trajTime(2)
 
    F = F4(t);
    pos = F * trajCoeff(1:5, 1:3);
 
elseif t <= trajTime(3)
 
    F = F3(t);
    pos = F * trajCoeff(6:9, 1:3);
 
elseif t <= trajTime(4)
 
    F = F3(t);
    pos = F * trajCoeff(10:13, 1:3);
 
else
 
    F = F4(t);
    pos = F * trajCoeff(14:18, 1:3);
 
end
 
% Konverter til meter
x = pos(1) / 1000;
y = pos(2) / 1000;
z = pos(3) / 1000;
 
end
 
 
function out = F4(t)
    out = [1, t, t^2, t^3, t^4];
end
 
function out = F3(t)
    out = [1, t, t^2, t^3];
end

== matlab function Simscape_model_Energy/MATLAB Function2 ==
  data: J5_angleDeg output; J5_angleRad input; J5_angleRef output
function [J5_angleDeg, J5_angleRef] = J5_angleCalc(J5_angleRad)

J5_angleDeg = rad2deg(J5_angleRad);

J5_angleRef = J5_angleRad;

if J5_angleRef > 180
    J5_angleRef = 180;
elseif J5_angleRef < 0;
    J5_angleRef = 0;
end

== matlab function Simscape_model_Energy/MATLAB Function3 ==
  data: rad input; deg output
function deg = radianToDegConversion(rad)

deg = rad2deg(rad);

== matlab function Simscape_model_Energy/MATLAB Function4 ==
  data: deg input; rad output
function rad = deg2rad(deg)

rad = deg2rad(deg);

== matlab function Simscape_model_Energy/MATLAB Function5 ==
  data: deg input; rad output
function rad = deg2rad(deg)

rad = deg2rad(deg);

== matlab function Simscape_model_Energy/MATLAB Function ==
  data: refX input; errX output; refY input; refZ input; sensX input; sensY input; sensZ input; errY output; errZ output; absErr output
function [errX, errY, errZ, absErr] = fcn(refX, refY, refZ, sensX, sensY, sensZ)
errX = refX - sensX;
errY = refY - sensY;
errZ = refZ - sensZ;

absErr = sqrt(errX^2 + errY^2 + errZ^2);

== matlab function Simscape_model_Energy/MATLAB Function6 ==
  data: rad input; deg output
function deg = radianToDegConversion(rad)

deg = rad2deg(rad);

== matlab function Simscape_model_Energy/Robot/LightBlue/MATLAB Function6 ==
  data: rad input; deg output
function deg = radianToDegConversion(rad)

deg = rad2deg(rad);

== matlab function Simscape_model_Energy/Subsystem/MATLAB Function7 ==
  data: torque input; P_motoring output; angularVelocity input; P_generating output
function [P_motoring, P_generating] = fcn(torque, angularVelocity)

if (torque <= 0 && angularVelocity < 0) || (torque >= 0 && angularVelocity > 0)
    P_motoring = torque * angularVelocity;
    P_generating = 0;
else
    P_generating = abs(torque * angularVelocity);
    P_motoring = 0;
end
